simulink model "Model_31_02_1"  (R2024b)
settings: Solver=FixedStepAuto  StartTime=0.0  StopTime=20  FixedStep=0.01  RelTol=1e-3
values from neighbouring files (symbols this model uses):
  b = pend1.b    [Code_31_02.m]
  c = pend1.c    [Code_31_02.m]
  F = -pend1.Kp*x_n_l_NL(:,3) - pend1.Kd * x_n_l_NL(:,4)    [Code_31_02.m]
  g = pend1.g    [Code_31_02.m]
  l = pend1.l    [Code_31_02.m]
  m = pend1.m    [Code_31_02.m]
  M = pend1.M    [Code_31_02.m]
settings Model: Creator=baron  LastModifiedBy=baron
settings DebuggingCC: AlgebraicLoopMsg=none

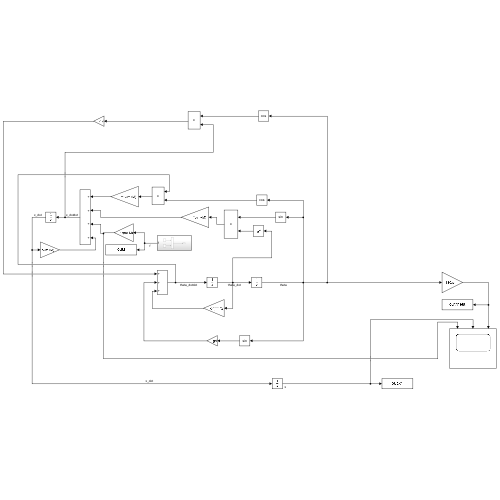
[thumbnail: Simulink's stored preview of the top-level diagram]
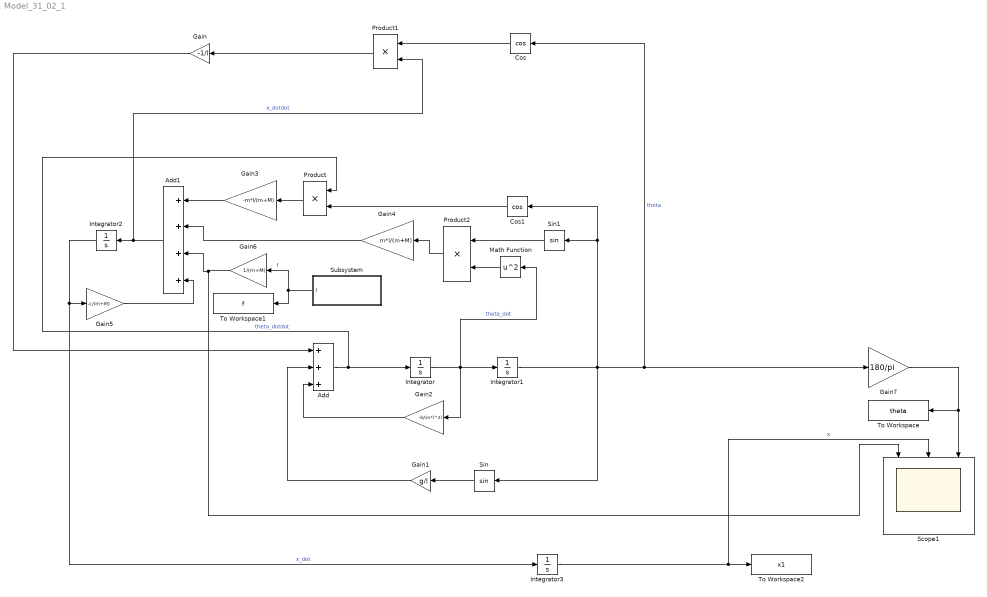
== system Model_31_02_1 ==
  Add : Sum  Inputs=+++
  Add1 : Sum  Inputs=++++
  Cos : Trigonometry  Operator=cos
  Cos1 : Trigonometry  Operator=cos
  Gain : Gain  Gain=-1/l
  Gain1 : Gain  Gain=g/l
  Gain2 : Gain  Gain=-b/(m*l^2)
  Gain3 : Gain  Gain=-m*l/(m+M)
  Gain4 : Gain  Gain=m*l/(m+M)
  Gain5 : Gain  Gain=-c/(m+M)
  Gain6 : Gain  Gain=1/(m+M)
  Gain7 : Gain  Gain=180/pi
  Integrator : Integrator
  Integrator1 : Integrator  InitialCondition=pi
  Integrator2 : Integrator
  Integrator3 : Integrator
  Math Function : Math  Operator=square
  Product : Product
  Product1 : Product
  Product2 : Product
  Scope1 : Scope  NumInputPorts=3
  Sin : Trigonometry
  Sin1 : Trigonometry
  Subsystem : Subsystem
  To Workspace : ToWorkspace  VariableName=theta  SampleTime=-1
  To Workspace1 : ToWorkspace  VariableName=f  SampleTime=-1
  To Workspace2 : ToWorkspace  VariableName=x1  SampleTime=-1
  wires:
  Integrator1/1 -> Sin1/1, Cos1/1, Gain7/1, Cos/1, Sin/1  "theta"
  Sin/1 -> Gain1/1
  Gain1/1 -> Add/2
  Integrator/1 -> Math Function/1, Gain2/1, Integrator1/1  "theta_dot"
  Add/1 -> Integrator/1, Product/1  "theta_dotdot"
  Cos/1 -> Product1/1
  Subsystem/1(f) -> Gain6/1, To Workspace1/1  "f"
  Gain2/1 -> Add/3
  Cos1/1 -> Product/2
  Product/1 -> Gain3/1
  Gain3/1 -> Add1/1
  Product1/1 -> Gain/1
  Math Function/1 -> Product2/2
  Sin1/1 -> Product2/1
  Product2/1 -> Gain4/1
  Gain4/1 -> Add1/2
  Add1/1 -> Product1/2, Integrator2/1  "x_dotdot"
  Integrator2/1 -> Integrator3/1, Gain5/1  "x_dot"
  Gain5/1 -> Add1/4
  Gain/1 -> Add/1
  Integrator3/1 -> To Workspace2/1, Scope1/2  "x"
  Gain7/1 -> Scope1/3, To Workspace/1
  Gain6/1 -> Scope1/1, Add1/3

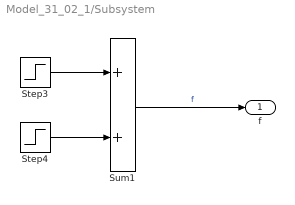
== system Model_31_02_1/Subsystem ==
  Step3 : Step  After=F  SampleTime=0
  Step4 : Step  Time=2  After=-F  SampleTime=0
  Sum1 : Sum
  f : Outport
  wires:
  Sum1/1 -> f/1  "f"
  Step4/1 -> Sum1/2
  Step3/1 -> Sum1/1
